simulink model "modele_freinage_regeneratif_v3"  (R2024a)
settings: Solver=VariableStepAuto  StartTime=0.0  StopTime=40  RelTol=1e-3
settings Model: Creator=HP  LastModifiedBy=HP

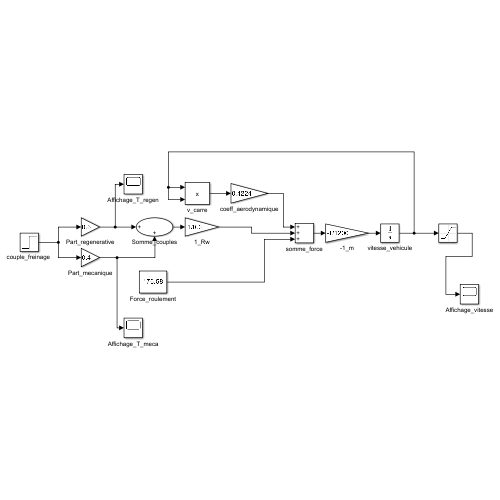
[thumbnail: Simulink's stored preview of the top-level diagram]
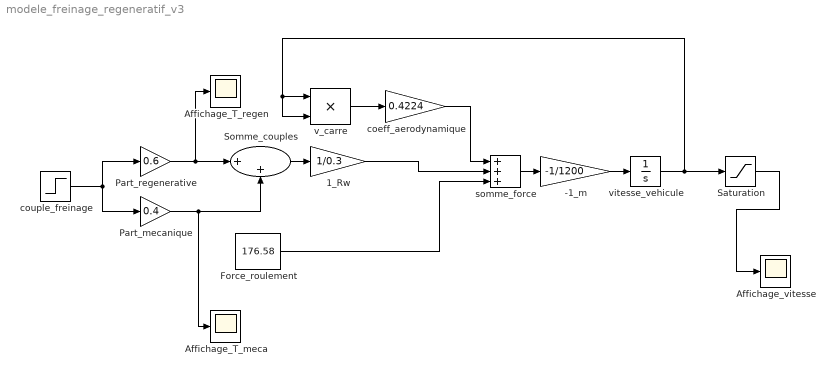
== system modele_freinage_regeneratif_v3 ==
  -1_m : Gain  Gain=-1/1200
  1_Rw : Gain  Gain=1/0.3
  Affichage_T_meca : Scope
  Affichage_T_regen : Scope
  Affichage_vitesse : Scope
  Force_roulement : Constant  Value=176.58
  Part_mecanique : Gain  Gain=0.4
  Part_regenerative : Gain  Gain=0.6
  Saturation : Saturate  UpperLimit=100  LowerLimit=0
  Somme_couples : Sum  Inputs=|++
  coeff_aerodynamique : Gain  Gain=0.4224
  "couple_freinage " : Step  After=150  SampleTime=0
  somme_force : Sum  Inputs=+++
  v_carre : Product
  vitesse_vehicule : Integrator  InitialCondition=20
  wires:
  somme_force/1 -> -1_m/1
  1_Rw/1 -> somme_force/2
  v_carre/1 -> coeff_aerodynamique/1
  coeff_aerodynamique/1 -> somme_force/1
  Force_roulement/1 -> somme_force/3
  vitesse_vehicule/1 -> Saturation/1, v_carre/2, v_carre/1
  -1_m/1 -> vitesse_vehicule/1
  Saturation/1 -> Affichage_vitesse/1
  "couple_freinage "/1 -> Part_regenerative/1, Part_mecanique/1
  Somme_couples/1 -> 1_Rw/1
  Part_regenerative/1 -> Affichage_T_regen/1, Somme_couples/1
  Part_mecanique/1 -> Affichage_T_meca/1, Somme_couples/2
